simulink model "commhdlQPSKTxRxLoopback"  (R2025b)
settings: Solver=FixedStepDiscrete  StartTime=0.0  StopTime=0.03  RelTol=1e-3
PostLoadFcn:
  | hScopeConfig = get_param([gcs '/Receiver/QPSK Rx/Frequency and Time Synchronizer/Symbol Synchronizer/No HDL/QPSK Receiver Eye Diagram'],'ScopeConfiguration');
  | 
  | hScopeConfig.OpenAtSimulationStart = false;
  | hScopeConfig.Visible = false;
  | SamplesPerSymbol = 4;
  | %UpsamplesRx = 1;
  | clear hScopeConfig
InitFcn:
  | % RxAlign decoder latency (flat_simfix): 41 = netlist value used for HDL; set
  | % rxAlignLat = 25 in the base workspace before a model-level simulation.
  | if ~exist('rxAlignLat','var'), rxAlignLat = uint16(41); end
  | commhdlQPSKTxRxModelInit;
  | % Rate bridge: ADRV9002/Jupiter radio runs at 15.36 MHz = 2x the 7.68 MHz
  | % (4 samples/symbol @ Rsym=1.92 MHz) the QPSK Rx requires. The deployed
  | % Receiver must downsample the ADC stream by 2. UpsamplesRx=1 fed the QPSK
  | % Rx 8 sps (2x-upsampled) and broke symbol sync / the loopback bit check.
  | UpsamplesRx = 1;   %% T8 RATE FIX: rail 15.36e6 == ADC bus rate,
  | %% no ingress decimation (was 2 when the rail sat on the 7.68e6 rung)
  | UpsamplesTx = 1;
  | clear simTimingOffset;
StopFcn:
  | if exist('simTimingOffset','var')
  |   disp('Simulation completed');
  |   %QPSKTxRxVerification;
  | end
undefined symbols (not defined in the file or in its folder): Add, Config, fsym, randsrc, RandStream, Rsym, rxAlignLat, Shift
libraries: hdlsllib x141, simulink x45, dspsigops x30, dsphdlfiltering2 x6, dsphdlsigops2 x4, dsphdlmathfun2 x4, commdigbbndpm3 x4, dspmlti4 x2, commchan3 x1, commrflib2 x1, commcnvcod2 x1
(part 6 of 9)

== system commhdlQPSKTxRxLoopback/Receiver/QPSK Rx/Frequency and Time Synchronizer/Phase Ambiguity Estimation and Correction/Phase Ambiguity Corrector/Reciprocal ==
  dataIn : Inport
  Compare To Constant : simulink/Logic and Bit Operations/Compare To Constant  relop=<  const=0  OutDataTypeStr=boolean
  Data Type Conversion : DataTypeConversion  OutDataTypeStr=fixdt(1,WL,0)  ConvertRealWorld=Stored Integer (SI)  SaturateOnIntegerOverflow=off  RndMeth=Floor
  Data Type Conversion1 : DataTypeConversion  OutDataTypeStr=fixdt(0,LUTAddrWL,0)  ConvertRealWorld=Stored Integer (SI)  SaturateOnIntegerOverflow=off  RndMeth=Floor
  Data Type Conversion2 : DataTypeConversion  OutDataTypeStr=fixdt(0,WL-LUTAddrWL,0)  ConvertRealWorld=Stored Integer (SI)  SaturateOnIntegerOverflow=off  RndMeth=Floor
  Delay : Delay  DelayLength=1
  Delay1 : Delay  DelayLength=1
  Delay2 : Delay  DelayLength=1
  Extract Bits : simulink/Logic and Bit Operations/Extract Bits  bitsToExtract=Range ending with least significant bit  numBits=LUTAddrWL  bitIdxRange=[0 7]  outScalingMode=Treat bit field as an integer
  Function Impl : Subsystem
  dataOut : Outport
  wires:
  dataIn/1 -> Data Type Conversion/1
  Extract Bits/1 -> Delay2/1
  Data Type Conversion/1 -> Delay/1
  Compare To Constant/1 -> Delay1/1
  Data Type Conversion1/1 -> Function Impl/2(LUTAddr)
  Function Impl/1(functionValues) -> dataOut/1
  Delay/1 -> Compare To Constant/1, Extract Bits/1
  Delay1/1 -> Data Type Conversion2/1
  Delay2/1 -> Data Type Conversion1/1
  Data Type Conversion2/1 -> Function Impl/1(switch)

== system commhdlQPSKTxRxLoopback/Receiver/QPSK Rx/Frequency and Time Synchronizer/Phase Ambiguity Estimation and Correction/Phase Ambiguity Estimator/Subsystem ==
  L : Inport
  H : Inport  Port=2
  Delay6 : Delay  DelayLength=1  InitialCondition=1
  Logical Operator : Logic  AllPortsSameDT=off  OutDataTypeStr=boolean
  Logical Operator1 : Logic  Operator=NOT  IconShape=distinctive  AllPortsSameDT=off  OutDataTypeStr=boolean
  Logical Operator2 : Logic  Operator=OR  AllPortsSameDT=off  OutDataTypeStr=boolean
  Out2 : Outport
  wires:
  L/1 -> Logical Operator1/1
  H/1 -> Logical Operator2/1
  Delay6/1 -> Out2/1, Logical Operator/2
  Logical Operator1/1 -> Logical Operator/1
  Logical Operator/1 -> Logical Operator2/2
  Logical Operator2/1 -> Delay6/1

== system commhdlQPSKTxRxLoopback/Receiver/QPSK Rx/Frequency and Time Synchronizer/Phase Ambiguity Estimation and Correction/Phase Ambiguity Estimator/Subsystem1 ==
  In1 : Inport
  validIn : Inport  Port=2
  Logical Operator1 : Logic  IconShape=distinctive  AllPortsSameDT=off  OutDataTypeStr=boolean
  Logical Operator2 : Logic  Operator=NOT  IconShape=distinctive  AllPortsSameDT=off  OutDataTypeStr=boolean
  validOut : Outport
  wires:
  In1/1 -> Logical Operator2/1
  validIn/1 -> Logical Operator1/2
  Logical Operator1/1 -> validOut/1
  Logical Operator2/1 -> Logical Operator1/1

== system commhdlQPSKTxRxLoopback/Receiver/QPSK Rx/Frequency and Time Synchronizer/Preamble Detector/Correlator/Magnitude Squared ==
  In1 : Inport
  Delay1 : Delay
  Delay2 : Delay
  Delay3 : Delay
  Math Function : Math  Operator=conj
  Product : Product
  Out1 : Outport
  wires:
  In1/1 -> Math Function/1, Delay2/1
  Math Function/1 -> Delay1/1
  Product/1 -> Delay3/1
  Delay2/1 -> Product/1
  Delay1/1 -> Product/2
  Delay3/1 -> Out1/1

== system commhdlQPSKTxRxLoopback/Receiver/QPSK Rx/Frequency and Time Synchronizer/Preamble Detector/Correlator/Magnitude Squared and Moving Sum ==
  scaled1 : Inport
  validIn : Inport  Port=2
  Add : Sum  Inputs=|+-  OutDataTypeStr=Inherit: Same as first input
  Add1 : Sum  Inputs=|++  OutDataTypeStr=Inherit: Same as first input
  Complex to Real-Imag1 : ComplexToRealImag  Output=Real
  Delay : Delay  DelayLength=26  ShowEnablePort=on
      settings: InputPortMap=u0,e6
  Delay{1..4,6,8..10,12} (9 alike) : Delay
  Delay11 : Delay  DelayLength=24
  Delay14 : Delay  DelayLength=1  ShowEnablePort=on
      settings: InputPortMap=u0,e6
  Delay5 : Delay  DelayLength=1
  Delay7 : Delay  DelayLength=1
  Gain : Gain  Gain=ThresoldGainFac  OutDataTypeStr=Inherit: Same as input
  Math Function1 : Math  Operator=conj
  Product1 : Product
  E1 : Outport
  wires:
  Add/1 -> Delay5/1
  validIn/1 -> Delay12/1
  Delay/1 -> Add/2
  Delay14/1 -> Add1/2
  Complex to Real-Imag1/1 -> Delay3/1
  Add1/1 -> Delay11/1, Delay14/1
  Delay11/1 -> E1/1
  scaled1/1 -> Delay6/1, Math Function1/1
  Math Function1/1 -> Delay1/1
  Product1/1 -> Delay2/1
  Gain/1 -> Delay4/1
  Delay6/1 -> Product1/1
  Delay1/1 -> Product1/2
  Delay2/1 -> Complex to Real-Imag1/1
  Delay3/1 -> Gain/1
  Delay4/1 -> Delay/1, Add/1
  Delay5/1 -> Add1/1
  Delay7/1 -> Delay14/2
  Delay8/1 -> Delay/2, Delay7/1
  Delay9/1 -> Delay8/1
  Delay10/1 -> Delay9/1
  Delay12/1 -> Delay10/1

== system commhdlQPSKTxRxLoopback/Receiver/QPSK Rx/Frequency and Time Synchronizer/Preamble Detector/FIFO/Validate Input Push Pop ==
  rst : Inport
  push : Inport  Port=2
  pop : Inport  Port=3
  Compare To Constant : hdlsllib/Logic and Bit Operations/Compare To Constant  relop===  const=0  OutDataTypeStr=boolean
  Compare To Constant1 : hdlsllib/Logic and Bit Operations/Compare To Constant  relop===  const=fifoSize  OutDataTypeStr=boolean
  Constant : Constant  Value=true  SampleTime=-1
  Constant1 : Constant  Value=false  SampleTime=-1
  Delay : Delay  DelayLength=1
  Logical Operator1 : Logic  Operator=XOR  AllPortsSameDT=off  OutDataTypeStr=boolean
  Logical Operator2 : Logic  Operator=NOT  AllPortsSameDT=off  OutDataTypeStr=boolean
  Logical Operator{3..5,7,9} (5 alike) : Logic  AllPortsSameDT=off  OutDataTypeStr=boolean
  Logical Operator6 : Logic  Operator=NOT  AllPortsSameDT=off  OutDataTypeStr=boolean
  Logical Operator8 : Logic  Operator=NOT  AllPortsSameDT=off  OutDataTypeStr=boolean
  MATLAB Function : MATLAB Function  TreatAsAtomicUnit=on  mask{initVal=0, countToVal=fifoSize}
      mask prompts: initVal "Initial value:"; countToVal "Count to value:"
  No HDL : Subsystem
  Switch : Switch  Criteria=u2 ~= 0  SaturateOnIntegerOverflow=off  InputSameDT=off
  valid push : Outport
  valid pop : Outport  Port=2
  numEntries : Outport  Port=3
  wires:
  Logical Operator9/1 -> Logical Operator1/1, valid push/1
  Logical Operator2/1 -> Logical Operator9/2
  Logical Operator5/1 -> Logical Operator4/1
  Logical Operator8/1 -> Logical Operator5/2
  push/1 -> Logical Operator5/1, Logical Operator9/1
  Logical Operator1/1 -> MATLAB Function/2(enb)
  Logical Operator6/1 -> Logical Operator7/2
  Logical Operator7/1 -> Switch/2, valid pop/1, Logical Operator8/1, Logical Operator1/2
  Compare To Constant1/1 -> Logical Operator4/2
  Constant/1 -> Switch/3
  Logical Operator4/1 -> No HDL/1(pushFullFIFO), Logical Operator2/1  "push on full FIFO"
  Logical Operator3/1 -> No HDL/2(popEmptyFIFO), Logical Operator6/1  "pop on empty FIFO"
  Constant1/1 -> Switch/1
  MATLAB Function/1(count) -> Delay/1
  Switch/1 -> MATLAB Function/3(dir)
  pop/1 -> Logical Operator3/2, Logical Operator7/1
  Compare To Constant/1 -> Logical Operator3/1
  rst/1 -> MATLAB Function/1(rst)
  Delay/1 -> Compare To Constant1/1, numEntries/1, Compare To Constant/1

== system commhdlQPSKTxRxLoopback/Receiver/QPSK Rx/Frequency and Time Synchronizer/Preamble Detector/Timing Adjust/No HDL ==
  note: This subsystem generates variables required for QPSKRxVerification for validation
  validIn : Inport
  timingOffset : Inport  Port=2
  syncPulse : Inport  Port=3
  Compare To Constant : simulink/Logic and Bit Operations/Compare To Constant  relop===  const=0  OutDataTypeStr=boolean
  Delay : Delay  DelayLength=4
  Delay1 : Delay  DelayLength=4
  Frame Counter : hdlsllib/Sources/HDL Counter  CountType=Free running  CountInit=0  CountStep=1  CountMax=bitsPerPacket/2 - 1  CountFromType=Initial value  CountFrom=0  CountResetPort=off  CountLoadPort=off  CountEnbPort=on  CountDirPort=off  CountHitOutputPort=off  CountDataType=Unsigned  CountWordLen=32  CountFracLen=0  CountSampTime=1
  Logical Operator : Logic  AllPortsSameDT=off  OutDataTypeStr=boolean
  No HDL : Subsystem
  No HDL1 : Subsystem
  Symbol Counter : hdlsllib/Sources/HDL Counter  CountType=Count limited  CountInit=0  CountStep=1  CountMax=bitsPerPacket/2 - 1  CountFromType=Initial value  CountFrom=0  CountResetPort=off  CountLoadPort=off  CountEnbPort=on  CountDirPort=off  CountHitOutputPort=off  CountDataType=Unsigned  CountWordLen=nextpow2(bitsPerPacket/2 - 1)  CountFracLen=0  CountSampTime=1
  Unit Delay Enabled Synchronous : hdlsllib/Discrete/Unit Delay Enabled Synchronous  InitialCondition=0.0  SampleTime=-1
  wires:
  timingOffset/1 -> Delay1/1
  validIn/1 -> Logical Operator/2, Symbol Counter/1
  Symbol Counter/1 -> Compare To Constant/1
  Logical Operator/1 -> Unit Delay Enabled Synchronous/2, Frame Counter/1
  Compare To Constant/1 -> Logical Operator/1
  Frame Counter/1 -> Unit Delay Enabled Synchronous/1
  syncPulse/1 -> Delay/1
  Unit Delay Enabled Synchronous/1 -> No HDL1/1(frameNumber)
  Delay/1 -> No HDL/Enable, No HDL1/Enable
  Delay1/1 -> No HDL/1(timingOffset)

== system commhdlQPSKTxRxLoopback/Receiver/QPSK Rx/Frequency and Time Synchronizer/Symbol Synchronizer/Gardner TED/GTED ==
  In1 : Inport
  Add : Sum
  Add1 : Sum  Inputs=+-
  Add2 : Sum  Inputs=+-
  Complex to Real-Imag : ComplexToRealImag
  Delay{,1,4..5,8,11} (6 alike) : Delay  DelayLength=1
  Delay{9..10,12..13} (4 alike) : Delay
  Product : Product
  Product1 : Product
  Out1 : Outport
  wires:
  Product/1 -> Delay10/1
  Product1/1 -> Delay13/1
  Add/1 -> Out1/1
  In1/1 -> Complex to Real-Imag/1
  Complex to Real-Imag/1 -> Add1/2, Delay/1
  Delay/1 -> Delay1/1
  Add1/1 -> Delay9/1
  Delay1/1 -> Delay8/1, Add1/1
  Delay5/1 -> Delay11/1, Add2/1
  Add2/1 -> Delay12/1
  Delay4/1 -> Delay5/1
  Complex to Real-Imag/2 -> Add2/2, Delay4/1
  Delay8/1 -> Product/1
  Delay9/1 -> Product/2
  Delay10/1 -> Add/1
  Delay11/1 -> Product1/1
  Delay12/1 -> Product1/2
  Delay13/1 -> Add/2

== system commhdlQPSKTxRxLoopback/Receiver/QPSK Rx/Frequency and Time Synchronizer/Symbol Synchronizer/No HDL/No HDL ==
  data : Inport
  Enable : EnablePort
  Data Type Conversion : DataTypeConversion  OutDataTypeStr=double  SaturateOnIntegerOverflow=off  RndMeth=Floor
  QPSK Receiver Constellation 1 : ConstellationDiagram  WindowPosition=[436.000000,110.000000,915.000000,708.000000,]  Visible=on  ScopeFrameLocation=window  SymbolsToDisplaySource=Property  SymbolsToDisplay=10000  Title=Before Symbol Synchronization  XLimits=[-1.9386 1.9401]  YLimits=[-1.9386 1.9401]  AxesLimits=[-1.9386 1.9401]  DefaultConfigurationName=comm.scopes.ConstellationDiagramBlockCfg
      settings: OpenAtSimulationStart=off
  To Workspace : ToWorkspace  VariableName=simBeforeSS  SampleTime=-1
      settings: Save2DSignal=2-D array (concatenate along first dimension)
  wires:
  Data Type Conversion/1 -> To Workspace/1, QPSK Receiver Constellation 1/1
  data/1 -> Data Type Conversion/1

== system commhdlQPSKTxRxLoopback/Receiver/QPSK Rx/Frequency and Time Synchronizer/Symbol Synchronizer/Rate Handle/FIFO ==
  in : Inport
  push : Inport  Port=2
  pop : Inport  Port=3
  reset : Inport  Port=4
  Delay1 : Delay  DelayLength=1
  Pop Counter : hdlsllib/Sources/HDL Counter  CountType=Count limited  CountInit=0  CountStep=1  CountMax=fifoSize -1  CountFromType=Initial value  CountFrom=0  CountResetPort=on  CountLoadPort=off  CountEnbPort=on  CountDirPort=off  CountHitOutputPort=off  CountDataType=Unsigned  CountWordLen=nextpow2(fifoSize)  CountFracLen=0  CountSampTime=1
  Push Counter : hdlsllib/Sources/HDL Counter  CountType=Count limited  CountInit=0  CountStep=1  CountMax=fifoSize -1  CountFromType=Initial value  CountFrom=0  CountResetPort=on  CountLoadPort=off  CountEnbPort=on  CountDirPort=off  CountHitOutputPort=off  CountDataType=Unsigned  CountWordLen=nextpow2(fifoSize)  CountFracLen=0  CountSampTime=1
  Simple Dual Port RAM : hdlsllib/HDL RAMs/Simple Dual Port RAM  ram_size=nextpow2(fifoSize)
  Validate Input Push Pop : Subsystem
  out : Outport
  numEntries : Outport  Port=2
  validPop : Outport  Port=3
  wires:
  Delay1/1 -> Push Counter/1, Pop Counter/1
  in/1 -> Simple Dual Port RAM/1
  reset/1 -> Validate Input Push Pop/1(rst), Delay1/1
  Validate Input Push Pop/2(valid pop) -> Pop Counter/2, validPop/1
  Validate Input Push Pop/1(valid push) -> Push Counter/2, Simple Dual Port RAM/3
  pop/1 -> Validate Input Push Pop/3(pop)
  push/1 -> Validate Input Push Pop/2(push)
  Pop Counter/1 -> Simple Dual Port RAM/4
  Push Counter/1 -> Simple Dual Port RAM/2
  Simple Dual Port RAM/1 -> out/1
  Validate Input Push Pop/3(numEntries) -> numEntries/1

== system commhdlQPSKTxRxLoopback/Transmitter/QPSK Tx/Bit Packetizer/Data Bits FIFO/No HDL/No HDL ==
  push : Inport
  full : Inport  Port=2
  ncount : Inport  Port=3
  empty : Inport  Port=4
  pop : Inport  Port=5
  Assertion : Assertion
  Assertion1 : Assertion
  Display : Display
  Logical Operator : Logic  Operator=NAND  AllPortsSameDT=off  OutDataTypeStr=boolean
  Logical Operator1 : Logic  Operator=NAND  AllPortsSameDT=off  OutDataTypeStr=boolean
  wires:
  Logical Operator1/1 -> Assertion1/1
  ncount/1 -> Display/1
  Logical Operator/1 -> Assertion/1
  pop/1 -> Logical Operator1/2
  full/1 -> Logical Operator/2
  empty/1 -> Logical Operator1/1
  push/1 -> Logical Operator/1

== system commhdlQPSKTxRxLoopback/TxRxComposite/Receiver/QPSK Rx/Frequency and Time Synchronizer/Carrier Synchronizer/Direct Digital Synthesis ==
  rst : Inport
  validIn : Inport  Port=2
  phaseInc : Inport  Port=3
  Data Type Conversion : DataTypeConversion  OutDataTypeStr=fixdt(1,21,21)  SaturateOnIntegerOverflow=off  RndMeth=Floor
  Data Type Conversion1 : DataTypeConversion  OutDataTypeStr=fixdt(1,21,0)  ConvertRealWorld=Stored Integer (SI)  SaturateOnIntegerOverflow=off  RndMeth=Floor
  Delay : Delay  DelayLength=1
  NCO : dsphdlsigops2/NCO  PhaseIncrementSource=Input port  PhaseIncrement=0  PhaseOffsetSource=Property  PhaseOffset=0  DitherSource=Property  NumDitherBits=11  SamplesPerFrame=1  LUTCompress=off  ResetAction=on  Waveform=Complex exponential  PhasePort=off  SimulateUsing=Code generation  AccumulatorWL=21  PhaseQuantization=on  NumQuantizerAccumulatorBits=14  OutputDataType=Binary point scaling  OutputWL=16  OutputFL=14
  Terminator : Terminator
  expOut : Outport
  wires:
  NCO/2 -> Terminator/1
  rst/1 -> NCO/2
  Data Type Conversion1/1 -> NCO/1
  NCO/1 -> expOut/1
  validIn/1 -> NCO/3
  Data Type Conversion/1 -> Data Type Conversion1/1
  Delay/1 -> Data Type Conversion/1
  phaseInc/1 -> Delay/1

== system commhdlQPSKTxRxLoopback/TxRxComposite/Receiver/QPSK Rx/Frequency and Time Synchronizer/Carrier Synchronizer/Loop Filter ==
  e : Inport
  validIn : Inport  Port=2
  internalRst : Inport  Port=3
  externalRst : Inport  Port=4
  cs_prop_gain : Inport  Port=5  OutDataTypeStr=uint32  SampleTime=1/(Rsym*SamplesPerSymbol)
  cs_integ_gain : Inport  Port=6  OutDataTypeStr=uint32  SampleTime=1/(Rsym*SamplesPerSymbol)
  Add : Sum  Inputs=+|+
  Add1 : Sum  Inputs=|++  OutDataTypeStr=Inherit: Same as first input
  Data Type Conversion1 : DataTypeConversion  OutDataTypeStr=fixdt(1,29,29)  SaturateOnIntegerOverflow=off  RndMeth=Floor
  Data Type Conversion2 : DataTypeConversion  OutDataTypeStr=fixdt(1,39,39)  SaturateOnIntegerOverflow=off  RndMeth=Floor
  Delay : Delay  DelayLength=1
  Delay{1..11,13} (12 alike) : Delay
  Delay12 : Delay  DelayLength=1
  Gain : Gain  Gain=fi(CSLoopFilterIntegGain/(2*pi),0,16,16)  ParamDataTypeStr=Inherit: Inherit from 'Gain'
  Gain1 : Gain  Gain=fi(CSLoopFilterPropGain/(2*pi),0,16,16)  ParamDataTypeStr=Inherit: Inherit from 'Gain'
  LGMux_cs_integ_gain : MATLAB Function  TreatAsAtomicUnit=on
  LGMux_cs_prop_gain : MATLAB Function  TreatAsAtomicUnit=on
  LGProd_cs_integ_gain : Product
  LGProd_cs_prop_gain : Product
  LGSw_cs_integ_gain : Switch  Criteria=u2 ~= 0
  LGSw_cs_prop_gain : Switch  Criteria=u2 ~= 0
  Logical Operator : Logic  Operator=OR  AllPortsSameDT=off  OutDataTypeStr=boolean
  Unit Delay Enabled Resettable Synchronous : hdlsllib/Discrete/Unit Delay Enabled Resettable Synchronous  InitialCondition=0.0  SampleTime=-1
  Unit Delay Enabled Resettable Synchronous1 : hdlsllib/Discrete/Unit Delay Enabled Resettable Synchronous  InitialCondition=0.0  SampleTime=-1
  v : Outport
  valid : Outport  Port=2
  rst : Outport  Port=3
  wires:
  Add/1 -> v/1
  Delay2/1 -> Add/1
  Add1/1 -> Unit Delay Enabled Resettable Synchronous1/1
  Unit Delay Enabled Resettable Synchronous1/1 -> Delay3/1, Add1/2
  Data Type Conversion2/1 -> Add1/1
  LGProd_cs_integ_gain/1 -> LGSw_cs_integ_gain/1
  Delay3/1 -> Add/2
  Gain/1 -> LGSw_cs_integ_gain/3
  Data Type Conversion1/1 -> Unit Delay Enabled Resettable Synchronous/1
  LGProd_cs_prop_gain/1 -> LGSw_cs_prop_gain/1
  Delay5/1 -> LGProd_cs_integ_gain/1, Gain/1
  LGMux_cs_integ_gain/2(nz) -> LGSw_cs_integ_gain/2
  Delay8/1 -> Delay4/1
  LGMux_cs_integ_gain/1(coeff) -> LGProd_cs_integ_gain/2
  LGSw_cs_integ_gain/1 -> Delay1/1
  Delay4/1 -> Delay/1, Unit Delay Enabled Resettable Synchronous1/2, Unit Delay Enabled Resettable Synchronous/2
  Delay12/1 -> Delay13/1
  LGMux_cs_prop_gain/1(coeff) -> LGProd_cs_prop_gain/2
  Unit Delay Enabled Resettable Synchronous/1 -> Delay2/1
  internalRst/1 -> Delay9/1
  cs_integ_gain/1 -> LGMux_cs_integ_gain/1(axi)
  Delay10/1 -> Delay12/1, Logical Operator/2
  Delay1/1 -> Data Type Conversion2/1
  LGMux_cs_prop_gain/2(nz) -> LGSw_cs_prop_gain/2
  Gain1/1 -> LGSw_cs_prop_gain/3
  cs_prop_gain/1 -> LGMux_cs_prop_gain/1(axi)
  externalRst/1 -> Logical Operator/1
  Delay13/1 -> rst/1
  Delay7/1 -> LGProd_cs_prop_gain/1, Gain1/1
  e/1 -> Delay7/1, Delay5/1
  Delay9/1 -> Delay10/1
  validIn/1 -> Delay8/1
  Delay11/1 -> valid/1
  Delay6/1 -> Data Type Conversion1/1
  LGSw_cs_prop_gain/1 -> Delay6/1
  Logical Operator/1 -> Unit Delay Enabled Resettable Synchronous/3, Unit Delay Enabled Resettable Synchronous1/3
  Delay/1 -> Delay11/1

== system commhdlQPSKTxRxLoopback/TxRxComposite/Receiver/QPSK Rx/Frequency and Time Synchronizer/Carrier Synchronizer/Phase Error Detector ==
  dataIn : Inport
  Add : Sum  Inputs=+|-
  Compare To Constant : simulink/Logic and Bit Operations/Compare To Constant  relop=>=  const=0  OutDataTypeStr=boolean
  Compare To Constant1 : simulink/Logic and Bit Operations/Compare To Constant  relop=>=  const=0  OutDataTypeStr=boolean
  Complex to Real-Imag : ComplexToRealImag
  Constant : Constant  OutDataTypeStr=fixdt(1,2,0)  SampleTime=1/(Rsym*SamplesPerSymbol)
  Constant1 : Constant  Value=-1  OutDataTypeStr=fixdt(1,2,0)  SampleTime=1/(Rsym*SamplesPerSymbol)
  Constant2 : Constant  OutDataTypeStr=fixdt(1,2,0)  SampleTime=1/(Rsym*SamplesPerSymbol)
  Constant3 : Constant  Value=-1  OutDataTypeStr=fixdt(1,2,0)  SampleTime=1/(Rsym*SamplesPerSymbol)
  Data Type Conversion3 : DataTypeConversion  OutDataTypeStr=fixdt(1,10+3,10)  SaturateOnIntegerOverflow=off  RndMeth=Floor
  Delay{,1..6} (7 alike) : Delay
  Product : Product
  Product1 : Product
  Switch : Switch  Threshold=1  SaturateOnIntegerOverflow=off  InputSameDT=off
  Switch1 : Switch  Threshold=1  SaturateOnIntegerOverflow=off  InputSameDT=off
  PhaseError : Outport
  wires:
  Delay6/1 -> Data Type Conversion3/1
  Add/1 -> Delay6/1
  Product1/1 -> Delay5/1
  Product/1 -> Delay4/1
  Delay3/1 -> Product1/2
  Delay5/1 -> Add/2
  dataIn/1 -> Complex to Real-Imag/1
  Constant/1 -> Switch/1
  Complex to Real-Imag/2 -> Compare To Constant1/1, Delay1/1
  Delay4/1 -> Add/1
  Compare To Constant/1 -> Switch/2
  Constant1/1 -> Switch/3
  Data Type Conversion3/1 -> PhaseError/1
  Delay/1 -> Product/1
  Delay1/1 -> Product/2
  Constant2/1 -> Switch1/1
  Compare To Constant1/1 -> Switch1/2
  Complex to Real-Imag/1 -> Compare To Constant/1, Delay2/1
  Constant3/1 -> Switch1/3
  Switch/1 -> Delay/1
  Delay2/1 -> Product1/1
  Switch1/1 -> Delay3/1

== system commhdlQPSKTxRxLoopback/TxRxComposite/Receiver/QPSK Rx/Frequency and Time Synchronizer/Coarse Frequency Compensator/CFO step change detector ==
  note: fixed point precision loss warning supressed for this subsystem
  In1 : Inport
  cfo_threshold : Inport  Port=2  OutDataTypeStr=uint32  SampleTime=1/(Rsym*SamplesPerSymbol)
  Add : Sum  Inputs=+-
  Compare To Constant : simulink/Logic and Bit Operations/Compare To Constant  relop=>  const=fi(CFOChangeDetectThreshold,1,22,21)  OutDataTypeStr=boolean
  Compare To Constant1 : simulink/Logic and Bit Operations/Compare To Constant  relop=<  const=fi(-CFOChangeDetectThreshold,1,22,21)  OutDataTypeStr=boolean
  Delay : Delay  DelayLength=6
  Delay1 : Delay  DelayLength=1
  LGMux_cfo_threshold : MATLAB Function  TreatAsAtomicUnit=on
  LGSw_cfo_threshold_1 : Switch  Criteria=u2 ~= 0
  LGSw_cfo_threshold_2 : Switch  Criteria=u2 ~= 0
  Logical Operator : Logic  Operator=OR  AllPortsSameDT=off  OutDataTypeStr=boolean
  Out1 : Outport
  wires:
  Logical Operator/1 -> Delay/1
  Delay/1 -> Out1/1
  LGSw_cfo_threshold_2/1 -> Logical Operator/2
  Compare To Constant/1 -> LGSw_cfo_threshold_1/3
  LGSw_cfo_threshold_1/1 -> Logical Operator/1
  LGMux_cfo_threshold/2(fireNeg) -> LGSw_cfo_threshold_2/1
  LGMux_cfo_threshold/1(firePos) -> LGSw_cfo_threshold_1/1
  Add/1 -> LGMux_cfo_threshold/2(x), Compare To Constant/1, Compare To Constant1/1
  cfo_threshold/1 -> LGMux_cfo_threshold/1(axi)
  Compare To Constant1/1 -> LGSw_cfo_threshold_2/3
  Delay1/1 -> Add/2
  LGMux_cfo_threshold/3(nz) -> LGSw_cfo_threshold_2/2, LGSw_cfo_threshold_1/2
  In1/1 -> Delay1/1, Add/1

== system commhdlQPSKTxRxLoopback/TxRxComposite/Receiver/QPSK Rx/Frequency and Time Synchronizer/Coarse Frequency Compensator/Coarse Frequency Estimator ==
  dataIn : Inport
  validIn : Inport  Port=2
  Delay{1,9..12} (5 alike) : Delay  DelayLength=1
  Delay{2..8} (7 alike) : Delay
  Extract Frequency : Subsystem
  Gain1 : Gain  Gain=1/integAvgLen  ParamDataTypeStr=fixdt(0,nextpow2(integAvgLen),nextpow2(integAvgLen))  OutDataTypeStr=Inherit: Same as input
  Integrator : Subsystem
  Math Function : Math  Operator=conj
  Product : Product
  Unit Delay Enabled Synchronous : hdlsllib/Discrete/Unit Delay Enabled Synchronous  InitialCondition=0.0  SampleTime=-1
  normFreqEst : Outport
  wires:
  Extract Frequency/1(normFreqOut) -> normFreqEst/1
  Delay11/1 -> Extract Frequency/2(validIn)
  Integrator/2(IntegValid) -> Delay11/1
  Delay2/1 -> Integrator/1(dataIn)
  Gain1/1 -> Delay2/1
  Delay5/1 -> Gain1/1
  dataIn/1 -> Unit Delay Enabled Synchronous/1, Delay1/1
  Delay10/1 -> Extract Frequency/1(datain)
  validIn/1 -> Unit Delay Enabled Synchronous/2, Delay9/1
  Unit Delay Enabled Synchronous/1 -> Delay12/1
  Delay1/1 -> Delay7/1
  Delay9/1 -> Delay6/1
  Math Function/1 -> Delay8/1
  Delay12/1 -> Math Function/1
  Product/1 -> Delay5/1
  Delay6/1 -> Delay3/1
  Delay7/1 -> Product/1
  Delay3/1 -> Delay4/1
  Delay8/1 -> Product/2
  Integrator/1(IntegOut) -> Delay10/1
  Delay4/1 -> Integrator/2(validIn)

== system commhdlQPSKTxRxLoopback/TxRxComposite/Receiver/QPSK Rx/Frequency and Time Synchronizer/Coarse Frequency Compensator/Raise Power to 4 ==
  dataIn : Inport
  validIn : Inport  Port=2
  Delay{1..8,11..12} (10 alike) : Delay
  Delay10 : Delay  DelayLength=1
  Delay9 : Delay  DelayLength=1
  Product1 : Product  OutDataTypeStr=Inherit: Same as first input
  Product2 : Product  OutDataTypeStr=Inherit: Same as first input
  dataOut : Outport
  validOut : Outport  Port=2
  wires:
  Delay12/1 -> validOut/1
  Delay10/1 -> Delay8/1
  Delay9/1 -> Delay6/1, Delay7/1
  validIn/1 -> Delay5/1
  Delay3/1 -> Product1/1
  Delay8/1 -> Delay12/1
  Delay4/1 -> Product1/2
  Delay11/1 -> dataOut/1
  Delay5/1 -> Delay2/1
  Product1/1 -> Delay1/1
  Delay2/1 -> Delay10/1
  Delay1/1 -> Delay9/1
  Delay6/1 -> Product2/1
  Product2/1 -> Delay11/1
  dataIn/1 -> Delay4/1, Delay3/1
  Delay7/1 -> Product2/2

== system commhdlQPSKTxRxLoopback/TxRxComposite/Receiver/QPSK Rx/Frequency and Time Synchronizer/No HDL/Subsystem ==
  In1 : Inport
  Enable : EnablePort

== system commhdlQPSKTxRxLoopback/TxRxComposite/Receiver/QPSK Rx/Frequency and Time Synchronizer/Packet Controller/End Generator ==
  validIn : Inport
  rst : Inport  Port=2
  Compare To Constant : simulink/Logic and Bit Operations/Compare To Constant  relop===  const=dataBitsPerPacket/2 - 1  OutDataTypeStr=boolean
  Delay6 : Delay  DelayLength=1
  HDL Counter : hdlsllib/Sources/HDL Counter  CountType=Count limited  CountInit=0  CountStep=1  CountMax=dataBitsPerPacket/2 - 1  CountFromType=Initial value  CountFrom=0  CountResetPort=on  CountLoadPort=off  CountEnbPort=on  CountDirPort=off  CountHitOutputPort=off  CountDataType=Unsigned  CountWordLen=nextpow2(dataBitsPerPacket/2 - 1)  CountFracLen=0  CountSampTime=1
  Logical Operator1 : Logic  IconShape=distinctive  AllPortsSameDT=off  OutDataTypeStr=boolean
  endOut : Outport
  wires:
  Delay6/1 -> endOut/1
  Logical Operator1/1 -> Delay6/1
  Compare To Constant/1 -> Logical Operator1/1
  HDL Counter/1 -> Compare To Constant/1
  validIn/1 -> HDL Counter/2, Logical Operator1/2
  rst/1 -> HDL Counter/1

== system commhdlQPSKTxRxLoopback/TxRxComposite/Receiver/QPSK Rx/Frequency and Time Synchronizer/Phase Ambiguity Estimation and Correction/Average Estimates ==
  endIn : Inport
  estin : Inport  Port=2
  validIn : Inport  Port=3
  Add : Sum  Inputs=++|
  Data Type Conversion : DataTypeConversion  OutDataTypeStr=fixdt(1,16+8,13)  SaturateOnIntegerOverflow=off  RndMeth=Floor
  Data Type Conversion1 : DataTypeConversion  OutDataTypeStr=fixdt(1,16+8,13)  SaturateOnIntegerOverflow=off  RndMeth=Floor
  Data Type Conversion2 : DataTypeConversion  OutDataTypeStr=fixdt(1,16,14)  SaturateOnIntegerOverflow=off  RndMeth=Floor
  Delay{,1..3} (4 alike) : Delay  DelayLength=1
  Divide by 8 : DataTypeConversion  OutDataTypeStr=fixdt(1,24,13+log2(8))  ConvertRealWorld=Stored Integer (SI)  SaturateOnIntegerOverflow=off  RndMeth=Floor
  Unit Delay Enabled Synchronous : hdlsllib/Discrete/Unit Delay Enabled Synchronous  InitialCondition=0.0  SampleTime=-1
  Unit Delay Enabled Resettable Synchronous : hdlsllib/Discrete/Unit Delay Enabled Resettable Synchronous  InitialCondition=0.0  SampleTime=-1
  avgEst : Outport
  wires:
  Data Type Conversion2/1 -> avgEst/1
  endIn/1 -> Delay2/1
  validIn/1 -> Delay1/1
  estin/1 -> Delay/1
  Divide by 8/1 -> Unit Delay Enabled Synchronous/1
  Delay2/1 -> Delay3/1, Unit Delay Enabled Synchronous/2
  Add/1 -> Data Type Conversion1/1
  Delay3/1 -> Unit Delay Enabled Resettable Synchronous/3
  Unit Delay Enabled Resettable Synchronous/1 -> Divide by 8/1, Add/1
  Delay/1 -> Data Type Conversion/1
  Delay1/1 -> Unit Delay Enabled Resettable Synchronous/2
  Data Type Conversion/1 -> Add/2
  Data Type Conversion1/1 -> Unit Delay Enabled Resettable Synchronous/1
  Unit Delay Enabled Synchronous/1 -> Data Type Conversion2/1

== system commhdlQPSKTxRxLoopback/TxRxComposite/Receiver/QPSK Rx/Frequency and Time Synchronizer/Phase Ambiguity Estimation and Correction/Phase Ambiguity Corrector ==
  note: Set this value to zero to disable phase ambiguity correction
  note: Let Z be the complex Phase Ambiguity estimate and Xbar be the data and X be the corrected data.
      | X = Xbar * conj(Z) * (1/abs(Z))
  dataIn : Inport
  estimate : Inport  Port=2
  validIn : Inport  Port=3
  Complex to Magnitude-Angle : dsphdlmathfun2/Complex to Magnitude-Angle  NumIterationsSource=Auto  NumIterations=10  OutputFormat=Magnitude  AngleFormat=Normalized  ScaleOutput=on  ScalingMethod=Shift-Add  SimulateUsing=Code generation
  Constant : Constant  OutDataTypeStr=boolean  SampleTime=-1
  Constant1 : Constant  OutMin=1  OutMax=1  OutDataTypeStr=boolean  SampleTime=-1
  Data Type Conversion : DataTypeConversion  OutDataTypeStr=fixdt(1,12,10)  SaturateOnIntegerOverflow=off  RndMeth=Floor
  Delay : Delay  DelayLength=15
  Delay1 : Delay  DelayLength=15
  Delay{2..4,7..8,10,13..18,22,25,28,36,38..39,41} (19 alike) : Delay  InitialCondition=0
  Delay11 : Delay  DelayLength=7  InitialCondition=0
  Delay12 : Delay  DelayLength=7  InitialCondition=0
  Delay5 : Delay  DelayLength=15
  Delay9 : Delay  DelayLength=7  InitialCondition=0
  Math Function : Math  Operator=conj  SignedPower=on  RndMeth=Zero
  Multiport Switch1 : MultiPortSwitch  DataPortOrder=Zero-based contiguous  Inputs=2  zeroidx=on  SaturateOnIntegerOverflow=off  InputSameDT=off
  Product1 : Product  OutDataTypeStr=Inherit: Same as first input
  Product2 : Product  OutDataTypeStr=Inherit: Same as first input
  Reciprocal : Subsystem  mask{WL=13, FL=10, outWL=26, Mapp=RAM - Based}
      mask prompts: WL "Input Word Length :"; FL "Input Fractional Length :"; outWL "Output Word Length :"; Mapp "Mapping Type:"
      mask init: same as commhdlQPSKTxRxLoopback/Receiver/QPSK Rx/Frequency and Time Synchronizer/Phase Ambiguity Estimation and Correction/Phase Ambiguity Corrector/Reciprocal
      mask TypeOptions Mapp: LUT - Based | RAM - Based
      mask DialogControl DescGroupVar Prompt: LUT - Based function
      mask DialogControl DescTextVar Prompt: This block is implemented for complex reciprocal
      mask Display: disp(['Reciprocal\n' get_param(gcb,'Mapp') '\nLatency = 7'])
  Terminator : Terminator
  dataOut : Outport
  validOut : Outport  Port=2
  wires:
  Multiport Switch1/1 -> dataOut/1
  Delay39/1 -> Multiport Switch1/3
  Constant/1 -> Multiport Switch1/1
  Delay41/1 -> Multiport Switch1/2
  Delay15/1 -> Product1/1
  Delay13/1 -> Delay41/1
  Complex to Magnitude-Angle/2 -> Terminator/1
  Delay11/1 -> Delay36/1
  dataIn/1 -> Delay/1
  validIn/1 -> Delay5/1
  Constant1/1 -> Complex to Magnitude-Angle/2
  Product1/1 -> Delay39/1
  Complex to Magnitude-Angle/1 -> Delay10/1
  Delay10/1 -> Reciprocal/1(dataIn)
  Delay7/1 -> Delay17/1
  estimate/1 -> Data Type Conversion/1
  Delay14/1 -> Delay16/1
  Product2/1 -> Delay4/1
  Delay17/1 -> Product1/2
  Delay12/1 -> Delay14/1
  Delay2/1 -> Delay12/1
  Delay/1 -> Delay8/1
  Delay8/1 -> Delay11/1
  Delay4/1 -> Delay15/1
  Delay25/1 -> Delay9/1
  Delay9/1 -> Math Function/1
  Reciprocal/1(dataOut) -> Delay3/1
  Math Function/1 -> Delay28/1
  Delay16/1 -> Delay18/1
  Delay3/1 -> Delay7/1
  Delay18/1 -> Delay22/1
  Delay38/1 -> Delay13/1
  Delay36/1 -> Product2/1, Delay38/1
  Data Type Conversion/1 -> Delay1/1, Complex to Magnitude-Angle/1
  Delay28/1 -> Product2/2
  Delay1/1 -> Delay25/1
  Delay5/1 -> Delay2/1
  Delay22/1 -> validOut/1

== system commhdlQPSKTxRxLoopback/TxRxComposite/Receiver/QPSK Rx/Frequency and Time Synchronizer/Phase Ambiguity Estimation and Correction/Phase Ambiguity Estimator ==
  dataIn : Inport
  syncPulse : Inport  Port=2
  validIn : Inport  Port=3
  Compare To Constant : simulink/Logic and Bit Operations/Compare To Constant  relop===  const=7  OutDataTypeStr=boolean
  Delay{1..3,8} (4 alike) : Delay  DelayLength=1
  Delay{4..7,9..11} (7 alike) : Delay
  Direct Lookup Table (n-D) : LookupNDDirect  NumberOfTableDimensions=1  Table=fi(preambleSymbols(3+1:3+8),1,16)  DiagnosticForOutOfRangeInput=Error
  HDL Counter : hdlsllib/Sources/HDL Counter  CountType=Count limited  CountInit=0  CountStep=1  CountMax=8-1  CountFromType=Initial value  CountFrom=0  CountResetPort=on  CountLoadPort=off  CountEnbPort=on  CountDirPort=off  CountHitOutputPort=off  CountDataType=Unsigned  CountWordLen=3  CountFracLen=0  CountSampTime=1
  Logical Operator : Logic  IconShape=distinctive  AllPortsSameDT=off  OutDataTypeStr=boolean
  Math Function : Math  Operator=conj  SignedPower=on  RndMeth=Zero
  Product : Product
  Subsystem : Subsystem
  Subsystem1 : Subsystem
  endOut : Outport
  estOut : Outport  Port=2
  validOut : Outport  Port=3
  wires:
  Delay9/1 -> estOut/1
  Delay11/1 -> endOut/1
  Delay4/1 -> Product/2
  Delay7/1 -> Delay11/1
  Math Function/1 -> Delay4/1
  Delay3/1 -> Delay7/1
  validIn/1 -> Subsystem1/2(validIn)
  Subsystem1/1(validOut) -> Delay2/1, HDL Counter/2, Logical Operator/1
  Direct Lookup Table (n-D)/1 -> Math Function/1
  Product/1 -> Delay9/1
  Delay2/1 -> Delay6/1
  syncPulse/1 -> Subsystem/1(L)
  Logical Operator/1 -> Delay3/1, Subsystem/2(H)
  Delay5/1 -> Product/1
  Delay1/1 -> Delay5/1
  HDL Counter/1 -> Delay8/1, Compare To Constant/1
  dataIn/1 -> Delay1/1
  Subsystem/1(Out2) -> HDL Counter/1, Subsystem1/1(In1)
  Delay6/1 -> Delay10/1
  Compare To Constant/1 -> Logical Operator/2
  Delay10/1 -> validOut/1
  Delay8/1 -> Direct Lookup Table (n-D)/1

== system commhdlQPSKTxRxLoopback/TxRxComposite/Receiver/QPSK Rx/Frequency and Time Synchronizer/Preamble Detector/Correlator ==
  dataIn : Inport
  validIn : Inport  Port=2
  Complex to Real-Imag : ComplexToRealImag  Output=Real
  Delay{1..6} (6 alike) : Delay  DelayLength=1
  Delay7 : Delay  DelayLength=4
  Delay8 : Delay  DelayLength=4
  Discrete FIR Filter : dsphdlfiltering2/Discrete FIR Filter  NumeratorSource=Property  Numerator=rxPreambleMFCoeffs  NumeratorPrototype=[]  FilterStructure=Direct form systolic  SerializationOption=Minimum number of cycles between valid input samples  NumCycles=2  NumberOfMultipliers=2  SimulateUsing=Code generation  roundingMode=Floor  overflowMode=off  CoefficientsDataTypeStr=Inherit: Same word length as input  OutputDataTypeStr=Inherit: Same word length as input  ResetInputPort=off  HDLGlobalReset=off  CoeffMultiplier=Multiplier  UseMultForPow2Coeff=on  FrameInputSymmOptim=off
  Magnitude Squared : Subsystem
  Magnitude Squared and Moving Sum : Subsystem
  ThresholdLimiter : MATLAB Function  TreatAsAtomicUnit=on
  dataOut : Outport
  threshold : Outport  Port=2
  validOut : Outport  Port=3
  wires:
  Delay8/1 -> Delay5/1
  Delay6/1 -> Magnitude Squared/1(In1)
  validIn/1 -> Magnitude Squared and Moving Sum/2(validIn), Discrete FIR Filter/2
  Delay2/1 -> dataOut/1
  Discrete FIR Filter/1 -> Delay6/1
  Discrete FIR Filter/2 -> Delay1/1
  Delay4/1 -> ThresholdLimiter/1(x)
  Magnitude Squared/1(Out1) -> Complex to Real-Imag/1
  Delay5/1 -> threshold/1
  Magnitude Squared and Moving Sum/1(E1) -> Delay4/1
  ThresholdLimiter/1(y) -> Delay8/1
  Delay1/1 -> Delay7/1
  dataIn/1 -> Magnitude Squared and Moving Sum/1(scaled1), Discrete FIR Filter/1
  Delay7/1 -> Delay3/1
  Delay3/1 -> validOut/1
  Complex to Real-Imag/1 -> Delay2/1

== system commhdlQPSKTxRxLoopback/TxRxComposite/Receiver/QPSK Rx/Frequency and Time Synchronizer/Preamble Detector/FIFO ==
  in : Inport
  push : Inport  Port=2
  pop : Inport  Port=3
  reset : Inport  Port=4
  Delay1 : Delay  DelayLength=1
  Pop Counter : hdlsllib/Sources/HDL Counter  CountType=Count limited  CountInit=0  CountStep=1  CountMax=fifoSize -1  CountFromType=Initial value  CountFrom=0  CountResetPort=on  CountLoadPort=off  CountEnbPort=on  CountDirPort=off  CountHitOutputPort=off  CountDataType=Unsigned  CountWordLen=nextpow2(fifoSize)  CountFracLen=0  CountSampTime=1
  Push Counter : hdlsllib/Sources/HDL Counter  CountType=Count limited  CountInit=0  CountStep=1  CountMax=fifoSize -1  CountFromType=Initial value  CountFrom=0  CountResetPort=on  CountLoadPort=off  CountEnbPort=on  CountDirPort=off  CountHitOutputPort=off  CountDataType=Unsigned  CountWordLen=nextpow2(fifoSize)  CountFracLen=0  CountSampTime=1
  Simple Dual Port RAM : hdlsllib/HDL RAMs/Simple Dual Port RAM  ram_size=nextpow2(fifoSize)
  Validate Input Push Pop : Subsystem
  out : Outport
  numEntries : Outport  Port=2
  validPop : Outport  Port=3
  wires:
  Pop Counter/1 -> Simple Dual Port RAM/4
  Simple Dual Port RAM/1 -> out/1
  Push Counter/1 -> Simple Dual Port RAM/2
  Validate Input Push Pop/3(numEntries) -> numEntries/1
  Validate Input Push Pop/1(valid push) -> Push Counter/2, Simple Dual Port RAM/3
  Delay1/1 -> Push Counter/1, Pop Counter/1
  Validate Input Push Pop/2(valid pop) -> Pop Counter/2, validPop/1
  pop/1 -> Validate Input Push Pop/3(pop)
  push/1 -> Validate Input Push Pop/2(push)
  in/1 -> Simple Dual Port RAM/1
  reset/1 -> Validate Input Push Pop/1(rst), Delay1/1

== system commhdlQPSKTxRxLoopback/TxRxComposite/Receiver/QPSK Rx/Frequency and Time Synchronizer/Preamble Detector/No HDL ==
  In1 : Inport
  In2 : Inport  Port=2
  Enable : EnablePort
  Data Type Conversion : DataTypeConversion  OutDataTypeStr=double  SaturateOnIntegerOverflow=off  RndMeth=Floor
  Data Type Conversion1 : DataTypeConversion  OutDataTypeStr=double  SaturateOnIntegerOverflow=off  RndMeth=Floor
  wires:
  Data Type Conversion/1 -> ?  "Correlation Value"
  In2/1 -> Data Type Conversion1/1
  In1/1 -> Data Type Conversion/1

== system commhdlQPSKTxRxLoopback/TxRxComposite/Receiver/QPSK Rx/Frequency and Time Synchronizer/Preamble Detector/Peak Search ==
  note: peak picker
  corr : Inport
  thresholdExceeded : Inport  Port=2
  validIn : Inport  Port=3
  Compare To Constant : simulink/Logic and Bit Operations/Compare To Constant  relop===  const=samplesPerFrame1x - 1  OutDataTypeStr=boolean
  Logical Operator : Logic  IconShape=distinctive  AllPortsSameDT=off  OutDataTypeStr=boolean
  Logical Operator4 : Logic  IconShape=distinctive  AllPortsSameDT=off  OutDataTypeStr=boolean
  Relational Operator : RelationalOperator  Operator=>  OutDataTypeStr=boolean  InputSameDT=off
  Terminator : Terminator
  Unit Delay Enabled Synchronous : hdlsllib/Discrete/Unit Delay Enabled Synchronous  InitialCondition=0.0  SampleTime=-1
  Unit Delay Enabled Synchronous1 : hdlsllib/Discrete/Unit Delay Enabled Synchronous  InitialCondition=0.0  SampleTime=-1
  Unit Delay Enabled Resettable Synchronous : hdlsllib/Discrete/Unit Delay Enabled Resettable Synchronous  InitialCondition=0.0  SampleTime=-1
  Unit Delay Enabled Resettable Synchronous1 : hdlsllib/Discrete/Unit Delay Enabled Resettable Synchronous  InitialCondition=0.0  SampleTime=-1
  timing Reference : hdlsllib/Sources/HDL Counter  CountType=Count limited  CountInit=0  CountStep=1  CountMax=samplesPerFrame1x - 1  CountFromType=Initial value  CountFrom=0  CountResetPort=off  CountLoadPort=off  CountEnbPort=on  CountDirPort=off  CountHitOutputPort=off  CountDataType=Unsigned  CountWordLen=nextpow2(samplesPerFrame1x - 1)  CountFracLen=0  CountSampTime=1
  timing Reference Long : hdlsllib/Sources/HDL Counter  CountType=Free running  CountInit=0  CountStep=1  CountMax=samplesPerFrame1x - 1  CountFromType=Initial value  CountFrom=0  CountResetPort=off  CountLoadPort=off  CountEnbPort=on  CountDirPort=off  CountHitOutputPort=off  CountDataType=Unsigned  CountWordLen=32  CountFracLen=0  CountSampTime=1
  timingOffset : Outport
  done : Outport  Port=2
  success : Outport  Port=3
  p1c_tref : Outport  Port=4
  p1c_treflong : Outport  Port=5
  p1c_runmax : Outport  Port=6
  p1c_newpk : Outport  Port=7
  p1c_heldts : Outport  Port=8
  wires:
  thresholdExceeded/1 -> Logical Operator4/2, Unit Delay Enabled Resettable Synchronous1/2, Unit Delay Enabled Resettable Synchronous1/1
  corr/1 -> Unit Delay Enabled Resettable Synchronous/1, Relational Operator/1
  Unit Delay Enabled Synchronous1/1 -> p1c_heldts/1, Terminator/1
  Unit Delay Enabled Synchronous/1 -> timingOffset/1
  Compare To Constant/1 -> Logical Operator/2
  timing Reference Long/1 -> p1c_treflong/1, Unit Delay Enabled Synchronous1/1
  validIn/1 -> timing Reference Long/1, timing Reference/1, Logical Operator/1
  Unit Delay Enabled Resettable Synchronous1/1 -> success/1
  Relational Operator/1 -> Logical Operator4/1
  Unit Delay Enabled Resettable Synchronous/1 -> p1c_runmax/1, Relational Operator/2
  Logical Operator/1 -> Unit Delay Enabled Resettable Synchronous/3, Unit Delay Enabled Resettable Synchronous1/3, done/1
  timing Reference/1 -> p1c_tref/1, Unit Delay Enabled Synchronous/1, Compare To Constant/1
  Logical Operator4/1 -> p1c_newpk/1, Unit Delay Enabled Synchronous1/2, Unit Delay Enabled Synchronous/2, Unit Delay Enabled Resettable Synchronous/2

== system commhdlQPSKTxRxLoopback/TxRxComposite/Receiver/QPSK Rx/Frequency and Time Synchronizer/Preamble Detector/Timing Adjust ==
  timingOffset : Inport
  timingOffsetValid : Inport  Port=2
  dataIn : Inport  Port=3
  validIn : Inport  Port=4
  Delay{,1..4} (5 alike) : Delay  DelayLength=1
  Logical Operator : Logic  AllPortsSameDT=off  OutDataTypeStr=boolean
  Logical Operator1 : Logic  Operator=NOT  AllPortsSameDT=off  OutDataTypeStr=boolean
  Logical Operator2 : Logic  Inputs=3  AllPortsSameDT=off  OutDataTypeStr=boolean
  No HDL : Subsystem
  Relational Operator : RelationalOperator  Operator===  OutDataTypeStr=boolean  InputSameDT=off
  State Register : hdlsllib/Discrete/Unit Delay Enabled Resettable Synchronous  InitialCondition=0.0  SampleTime=-1
  Unit Delay Enabled Synchronous3 : hdlsllib/Discrete/Unit Delay Enabled Synchronous  InitialCondition=0.0  SampleTime=-1
  timing Reference : hdlsllib/Sources/HDL Counter  CountType=Count limited  CountInit=0  CountStep=1  CountMax=searchSamples - 1  CountFromType=Initial value  CountFrom=0  CountResetPort=off  CountLoadPort=off  CountEnbPort=on  CountDirPort=off  CountHitOutputPort=off  CountDataType=Unsigned  CountWordLen=nextpow2(searchSamples - 1)  CountFracLen=0  CountSampTime=1
  dataOut : Outport
  validOut : Outport  Port=2
  SyncPulse : Outport  Port=3
  p1c_armed : Outport  Port=4
  p1c_taref : Outport  Port=5
  p1c_accoff : Outport  Port=6
  wires:
  Delay/1 -> SyncPulse/1
  Logical Operator2/1 -> No HDL/3(syncPulse), Delay/1, Delay2/1
  Unit Delay Enabled Synchronous3/1 -> p1c_accoff/1, Relational Operator/2
  Logical Operator1/1 -> Logical Operator/2
  validIn/1 -> timing Reference/1, Logical Operator2/1, Delay3/1, No HDL/1(validIn)
  Delay4/1 -> dataOut/1
  Delay1/1 -> Logical Operator1/1
  Relational Operator/1 -> Logical Operator2/2
  timingOffset/1 -> Unit Delay Enabled Synchronous3/1
  timingOffsetValid/1 -> State Register/2, State Register/1, Unit Delay Enabled Synchronous3/2, Logical Operator/1
  Delay3/1 -> validOut/1
  State Register/1 -> p1c_armed/1, Logical Operator2/3, Delay1/1
  dataIn/1 -> Delay4/1
  timing Reference/1 -> p1c_taref/1, Relational Operator/1, No HDL/2(timingOffset)
  Delay2/1 -> State Register/3

== system commhdlQPSKTxRxLoopback/TxRxComposite/Receiver/QPSK Rx/Frequency and Time Synchronizer/Symbol Synchronizer/Gardner TED ==
  data : Inport
  strobe : Inport  Port=2
  Constant : Constant  Value=0  OutDataTypeStr=Inherit: Inherit via back propagation  SampleTime=1/(Rsym*SamplesPerSymbol)
  Delay10 : Delay  DelayLength=4
  GTED : Subsystem
  Switch : Switch  Criteria=u2 ~= 0  InputSameDT=off
  e : Outport  VectorParamsAs1DForOutWhenUnconnected=off
  wires:
  Constant/1 -> Switch/3
  Delay10/1 -> Switch/2
  GTED/1(Out1) -> Switch/1
  Switch/1 -> e/1
  strobe/1 -> Delay10/1
  data/1 -> GTED/1(In1)

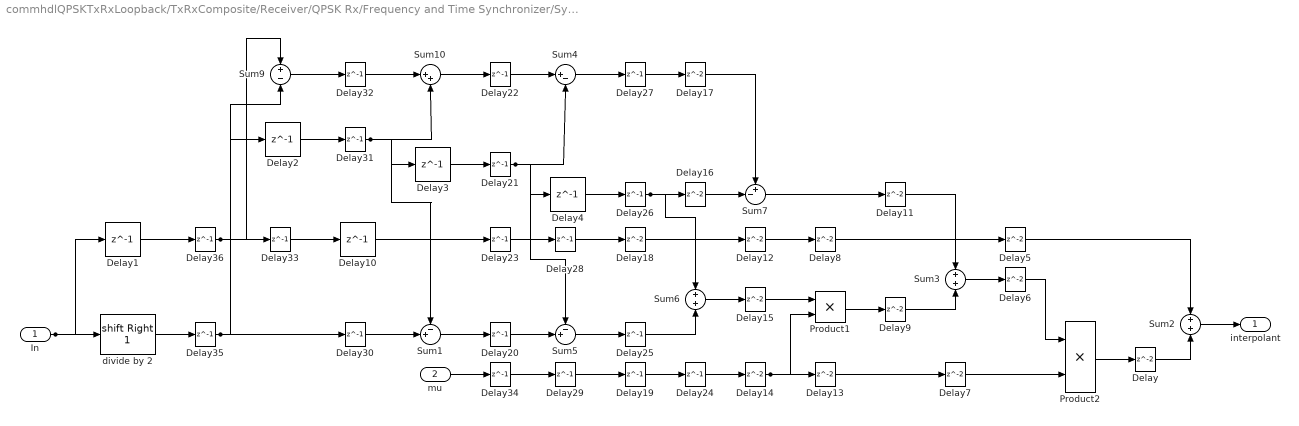
== system commhdlQPSKTxRxLoopback/TxRxComposite/Receiver/QPSK Rx/Frequency and Time Synchronizer/Symbol Synchronizer/Interpolation Filter ==
  In : Inport
  mu : Inport  Port=2
  Delay{,5..9,11..18} (14 alike) : Delay
  Delay{1..4,10} (5 alike) : Delay  DelayLength=1  InitialCondition=0
  Delay{19..36} (18 alike) : Delay  DelayLength=1
  Product1 : Product  OutDataTypeStr=fixdt(1,16,10)  RndMeth=Zero
  Product2 : Product  RndMeth=Zero  OutDataTypeStr=Inherit: Same as first input
  Sum1 : Sum  Inputs=-+|
  Sum10 : Sum  Inputs=|++
  Sum2 : Sum  Inputs=+|+
  Sum3 : Sum  Inputs=+|+  OutDataTypeStr=fixdt(1,16,10)
  Sum4 : Sum  Inputs=|+-
  Sum5 : Sum  Inputs=-+|
  Sum6 : Sum  Inputs=+|+  OutDataTypeStr=fixdt(1,16,11)  SaturateOnIntegerOverflow=on
  Sum7 : Sum  Inputs=+-|  OutDataTypeStr=fixdt(1,16,10)
  Sum9 : Sum  Inputs=+-
  divide by 2 : ArithShift  BitShiftNumber=1  BitShiftDirection=Right
  interpolant : Outport
  wires:
  Delay/1 -> Sum2/2
  Product2/1 -> Delay/1
  Delay6/1 -> Product2/1
  Delay5/1 -> Sum2/1
  Delay7/1 -> Product2/2
  Sum3/1 -> Delay6/1
  Delay11/1 -> Sum3/1
  Delay15/1 -> Product1/1
  Delay12/1 -> Delay8/1
  Delay14/1 -> Delay13/1, Product1/2
  Sum7/1 -> Delay11/1
  Delay24/1 -> Delay14/1
  Delay17/1 -> Sum7/1
  Product1/1 -> Delay9/1
  Delay25/1 -> Sum6/2
  Delay30/1 -> Sum1/2
  Delay1/1 -> Delay36/1
  Sum6/1 -> Delay15/1
  Delay19/1 -> Delay24/1
  Sum9/1 -> Delay32/1
  Delay31/1 -> Delay3/1, Sum10/2, Sum1/1
  Delay35/1 -> Delay2/1, Delay30/1, Sum9/2
  Delay2/1 -> Delay31/1
  Sum2/1 -> interpolant/1
  Delay26/1 -> Delay16/1, Sum6/1
  Delay23/1 -> Delay28/1
  Delay29/1 -> Delay19/1
  Delay36/1 -> Delay33/1, Sum9/1
  Sum5/1 -> Delay25/1
  divide by 2/1 -> Delay35/1
  Delay20/1 -> Sum5/2
  Delay8/1 -> Delay5/1
  Sum10/1 -> Delay22/1
  In/1 -> divide by 2/1, Delay1/1
  Delay3/1 -> Delay21/1
  Delay32/1 -> Sum10/1
  Sum1/1 -> Delay20/1
  Delay33/1 -> Delay10/1
  Sum4/1 -> Delay27/1
  Delay9/1 -> Sum3/2
  Delay16/1 -> Sum7/2
  Delay28/1 -> Delay18/1
  mu/1 -> Delay34/1
  Delay22/1 -> Sum4/1
  Delay21/1 -> Delay4/1, Sum5/1, Sum4/2
  Delay10/1 -> Delay23/1
  Delay34/1 -> Delay29/1
  Delay13/1 -> Delay7/1
  Delay4/1 -> Delay26/1
  Delay27/1 -> Delay17/1
  Delay18/1 -> Delay12/1

== system commhdlQPSKTxRxLoopback/TxRxComposite/Receiver/QPSK Rx/Frequency and Time Synchronizer/Symbol Synchronizer/Loop Filter ==
  note: Proportional-Plus-Integrator Loop Filter,
      | Infinite DC Response to guarantee convergence
  e : Inport
  ss_prop_gain : Inport  Port=2  OutDataTypeStr=uint32  SampleTime=1/(Rsym*SamplesPerSymbol)
  ss_integ_gain : Inport  Port=3  OutDataTypeStr=uint32  SampleTime=1/(Rsym*SamplesPerSymbol)
  Add : Sum
  Add2 : Sum  Inputs=|++  OutDataTypeStr=Inherit: Same as first input
  Data Type Conversion17 : DataTypeConversion  OutDataTypeStr=fixdt(1,11,10)  RndMeth=Floor
  Delay : Delay  DelayLength=1
  Delay1 : Delay  DelayLength=1  InitialCondition=0
  Delay2 : Delay  InitialCondition=0
  Delay3 : Delay  InitialCondition=0
  Delay4 : Delay  DelayLength=1  InitialCondition=0
  Delay5 : Delay  InitialCondition=0
  Delay6 : Delay  DelayLength=1
  IntegClamp : Saturate  UpperLimit=0.06  LowerLimit=-0.06
  K1 : Gain  Gain=fi(SSLoopFilterPropGain,1,24,24)  ParamDataTypeStr=Inherit: Inherit from 'Gain'  OutDataTypeStr=fixdt(1,30,23)
  K2 : Gain  Gain=fi(SSLoopFilterIntegGain,1,24,24)  ParamDataTypeStr=Inherit: Inherit from 'Gain'  OutDataTypeStr=fixdt(1,30,23)
  LGMux_ss_integ_gain : MATLAB Function  TreatAsAtomicUnit=on
  LGMux_ss_prop_gain : MATLAB Function  TreatAsAtomicUnit=on
  LGProd_ss_integ_gain : Product  OutDataTypeStr=fixdt(1,30,23)
  LGProd_ss_prop_gain : Product  OutDataTypeStr=fixdt(1,30,23)
  LGSw_ss_integ_gain : Switch  Criteria=u2 ~= 0  OutDataTypeStr=fixdt(1,30,23)
  LGSw_ss_prop_gain : Switch  Criteria=u2 ~= 0  OutDataTypeStr=fixdt(1,30,23)
  v : Outport
  wires:
  Data Type Conversion17/1 -> v/1
  Add/1 -> Data Type Conversion17/1
  Delay4/1 -> Add/2
  IntegClamp/1 -> Delay4/1, Delay/1
  Delay1/1 -> Add/1
  Delay5/1 -> Delay6/1
  LGSw_ss_integ_gain/1 -> Delay5/1
  Delay6/1 -> Add2/1
  ss_prop_gain/1 -> LGMux_ss_prop_gain/1(axi)
  K2/1 -> LGSw_ss_integ_gain/3
  Delay3/1 -> Delay1/1
  LGSw_ss_prop_gain/1 -> Delay3/1
  e/1 -> Delay2/1
  LGMux_ss_prop_gain/1(coeff) -> LGProd_ss_prop_gain/2
  LGMux_ss_prop_gain/2(nz) -> LGSw_ss_prop_gain/2
  Delay2/1 -> LGProd_ss_integ_gain/1, LGProd_ss_prop_gain/1, K1/1, K2/1
  ss_integ_gain/1 -> LGMux_ss_integ_gain/1(axi)
  LGMux_ss_integ_gain/1(coeff) -> LGProd_ss_integ_gain/2
  LGProd_ss_prop_gain/1 -> LGSw_ss_prop_gain/1
  Delay/1 -> Add2/2
  LGMux_ss_integ_gain/2(nz) -> LGSw_ss_integ_gain/2
  K1/1 -> LGSw_ss_prop_gain/3
  Add2/1 -> IntegClamp/1
  LGProd_ss_integ_gain/1 -> LGSw_ss_integ_gain/1

== system commhdlQPSKTxRxLoopback/TxRxComposite/Receiver/QPSK Rx/Frequency and Time Synchronizer/Symbol Synchronizer/No HDL ==
  data : Inport
  valid : Inport  Port=2
  Data Type Conversion : DataTypeConversion  OutDataTypeStr=double  SaturateOnIntegerOverflow=off  RndMeth=Floor
  No HDL : Subsystem
  QPSK Receiver Eye Diagram : EyeDiagramBlock  WindowPosition=[403.000000,370.000000,417.000000,506.000000,]  ScopeFrameLocation=window  SamplesPerSymbol=SamplesPerSymbol  SymbolsPerTrace=1  Title=RRC Matched Filtered Output  YLimits=[-1.1602,1.2629]
      settings: OpenAtSimulationStart=off
  Unit Delay Enabled Synchronous : hdlsllib/Discrete/Unit Delay Enabled Synchronous  InitialCondition=0.0  SampleTime=-1
  wires:
  Data Type Conversion/1 -> QPSK Receiver Eye Diagram/1
  Unit Delay Enabled Synchronous/1 -> Data Type Conversion/1
  valid/1 -> Unit Delay Enabled Synchronous/2, No HDL/Enable
  data/1 -> No HDL/1(data), Unit Delay Enabled Synchronous/1
